simulink model "sens_acq_imu"  (R2026b)
settings: Solver=VariableStepAuto
values from neighbouring files (symbols this model uses):
  P = (P + P.')/2    [sens_nav_ekf.m]
undefined symbols (not defined in the file or in its folder): Ts
libraries: simulink x6
settings Model: Creator=aomar  LastModifiedBy=aomar

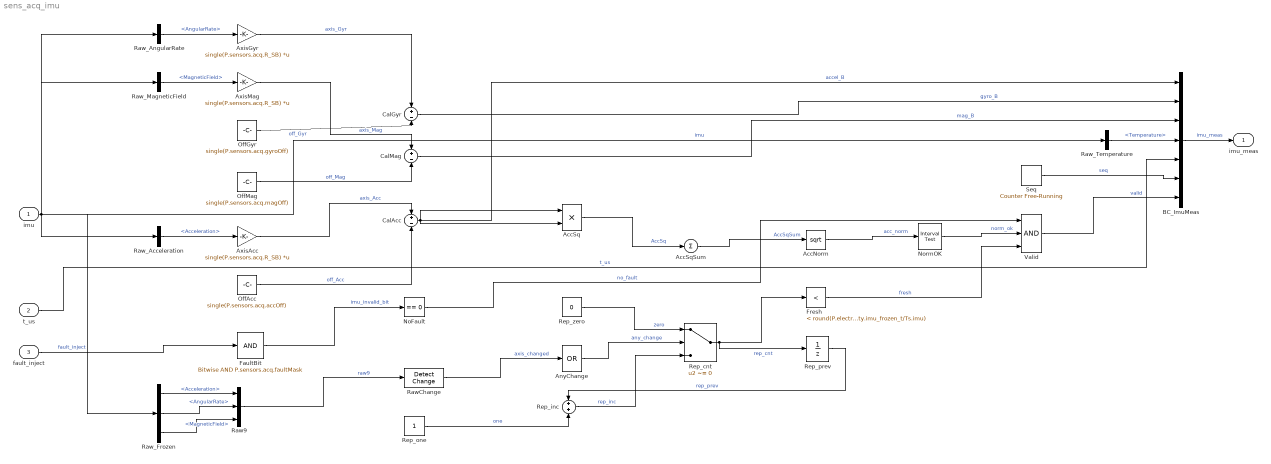
== system sens_acq_imu ==
  imu : Inport  OutDataTypeStr=Bus: Bus_ImuRaw  SampleTime=Ts.imu
  t_us : Inport  Port=2  OutDataTypeStr=uint32  PortDimensions=1  SampleTime=Ts.imu
  fault_inject : Inport  Port=3  OutDataTypeStr=uint32  PortDimensions=1  SampleTime=Ts.imu
  AccNorm : Sqrt
  AccSq : Product  Inputs=**
  AccSqSum : Sum  Inputs=+
  AnyChange : Logic  Operator=OR  Inputs=1  AllPortsSameDT=off  OutDataTypeStr=boolean
  AxisAcc : Gain  Gain=single(P.sensors.acq.R_SB)  Multiplication=Matrix(K*u)  OutDataTypeStr=Inherit: Same as input  ParamDataTypeStr=Inherit: Same as input
  AxisGyr : Gain  Gain=single(P.sensors.acq.R_SB)  Multiplication=Matrix(K*u)  OutDataTypeStr=Inherit: Same as input  ParamDataTypeStr=Inherit: Same as input
  AxisMag : Gain  Gain=single(P.sensors.acq.R_SB)  Multiplication=Matrix(K*u)  OutDataTypeStr=Inherit: Same as input  ParamDataTypeStr=Inherit: Same as input
  BC_ImuMeas : BusCreator  Inputs=7  OutDataTypeStr=Bus: Bus_ImuMeas  NonVirtualBus=on
      settings: InheritFromInputs=off
  CalAcc : Sum  Inputs=+-  OutDataTypeStr=Inherit: Same as first input
  CalGyr : Sum  Inputs=+-  OutDataTypeStr=Inherit: Same as first input
  CalMag : Sum  Inputs=+-  OutDataTypeStr=Inherit: Same as first input
  FaultBit : simulink/Logic and Bit Operations/Bitwise Operator  logicop=AND  UseBitMask=on  BitMask=P.sensors.acq.faultMask  BitMaskRealWorld=Stored Integer
  Fresh : simulink/Logic and Bit Operations/Compare To Constant  relop=<  const=round(P.electronics.safety.imu_frozen_t/Ts.imu)  OutDataTypeStr=boolean
  NoFault : simulink/Logic and Bit Operations/Compare To Zero  relop===  OutDataTypeStr=boolean
  NormOK : simulink/Logic and Bit Operations/Interval Test  IntervalClosedRight=on  uplimit=P.sensors.acq.accNormRange(2)  IntervalClosedLeft=on  lowlimit=P.sensors.acq.accNormRange(1)  OutDataTypeStr=boolean
  OffAcc : Constant  Value=single(P.sensors.acq.accOff)  OutDataTypeStr=single
  OffGyr : Constant  Value=single(P.sensors.acq.gyroOff)  OutDataTypeStr=single
  OffMag : Constant  Value=single(P.sensors.acq.magOff)  OutDataTypeStr=single
  Raw9 : Concatenate  NumInputs=3
  RawChange : simulink/Logic and Bit Operations/Detect Change  vinit=0  OutDataTypeStr=boolean
  Raw_Acceleration : BusSelector  OutputSignals=Acceleration
  Raw_AngularRate : BusSelector  OutputSignals=AngularRate
  Raw_Frozen : BusSelector  OutputSignals=Acceleration,AngularRate,MagneticField
  Raw_MagneticField : BusSelector  OutputSignals=MagneticField
  Raw_Temperature : BusSelector  OutputSignals=Temperature
  Rep_cnt : Switch  Criteria=u2 ~= 0  SaturateOnIntegerOverflow=off  InputSameDT=off
  Rep_inc : Sum  OutDataTypeStr=uint16  SaturateOnIntegerOverflow=on
  Rep_one : Constant  OutDataTypeStr=uint16
  Rep_prev : UnitDelay  SampleTime=Ts.imu
  Rep_zero : Constant  Value=0  OutDataTypeStr=uint16
  Seq : simulink/Sources/Counter Free-Running  NumBits=16  tsamp=Ts.imu
  Valid : Logic  Inputs=3  AllPortsSameDT=off  OutDataTypeStr=boolean
  imu_meas : Outport  OutDataTypeStr=Bus: Bus_ImuMeas
  wires:
  imu/1 -> Raw_Frozen/1, Raw_AngularRate/1, Raw_MagneticField/1, Raw_Temperature/1, Raw_Acceleration/1  "imu"
  t_us/1 -> BC_ImuMeas/5  "t_us"
  fault_inject/1 -> FaultBit/1  "fault_inject"
  Raw_AngularRate/1 -> AxisGyr/1  "<AngularRate>"
  Raw_MagneticField/1 -> AxisMag/1  "<MagneticField>"
  Raw_Acceleration/1 -> AxisAcc/1  "<Acceleration>"
  Raw_Frozen/1 -> Raw9/1  "<Acceleration>"
  Raw_Frozen/2 -> Raw9/2  "<AngularRate>"
  Raw_Frozen/3 -> Raw9/3  "<MagneticField>"
  Raw9/1 -> RawChange/1  "raw9"
  AxisGyr/1 -> CalGyr/1  "axis_Gyr"
  AxisMag/1 -> CalMag/1  "axis_Mag"
  OffGyr/1 -> CalGyr/2  "off_Gyr"
  OffMag/1 -> CalMag/2  "off_Mag"
  AxisAcc/1 -> CalAcc/1  "axis_Acc"
  OffAcc/1 -> CalAcc/2  "off_Acc"
  FaultBit/1 -> NoFault/1  "imu_invalid_bit"
  CalGyr/1 -> BC_ImuMeas/2  "gyro_B"
  CalMag/1 -> BC_ImuMeas/3  "mag_B"
  CalAcc/1 -> BC_ImuMeas/1, AccSq/1, AccSq/2  "accel_B"
  NoFault/1 -> Valid/1  "no_fault"
  Rep_one/1 -> Rep_inc/2  "one"
  RawChange/1 -> AnyChange/1  "axis_changed"
  Rep_inc/1 -> Rep_cnt/3  "rep_inc"
  AccSq/1 -> AccSqSum/1  "AccSq"
  Rep_zero/1 -> Rep_cnt/1  "zero"
  AnyChange/1 -> Rep_cnt/2  "any_change"
  AccSqSum/1 -> AccNorm/1  "AccSqSum"
  Rep_cnt/1 -> Fresh/1, Rep_prev/1  "rep_cnt"
  AccNorm/1 -> NormOK/1  "acc_norm"
  Fresh/1 -> Valid/3  "fresh"
  Rep_prev/1 -> Rep_inc/1  "rep_prev"
  NormOK/1 -> Valid/2  "norm_ok"
  Seq/1 -> BC_ImuMeas/6  "seq"
  Valid/1 -> BC_ImuMeas/7  "valid"
  Raw_Temperature/1 -> BC_ImuMeas/4  "<Temperature>"
  BC_ImuMeas/1 -> imu_meas/1  "imu_meas"
